simulink library "environmentLibrary"  (R2026a)
settings: Solver=ode45  EnableMultiTasking=on
undefined symbols (not defined in the file): decyear, initDate, leapyear
libraries: aerolibatmos2 x1, aerolibgravity2 x1
settings Model: Creator=The MathWorks, Inc.  LastModifiedBy=The MathWorks, Inc.
settings HardwareCC: ProdHWDeviceType=32-bit Generic

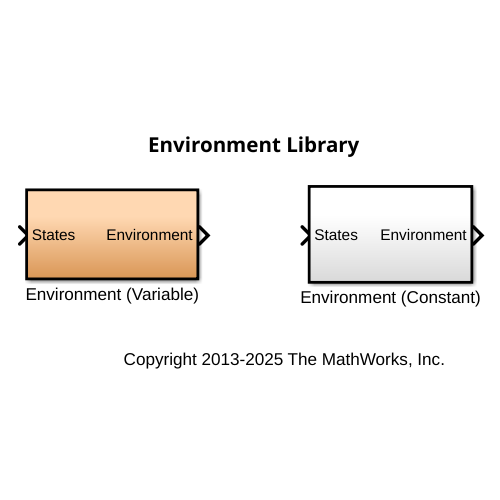
[thumbnail: Simulink's stored preview of the top-level diagram]
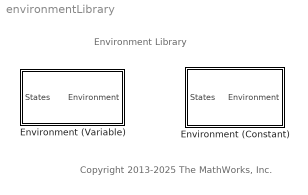
== system environmentLibrary ==
  note: Copyright 2013-2025 The MathWorks, Inc.
  note: Environment Library
  Environment (Constant) : Subsystem  TreatAsAtomicUnit=on
  Environment (Variable) : Subsystem  TreatAsAtomicUnit=on  VariantControl=Variants.Environment==1

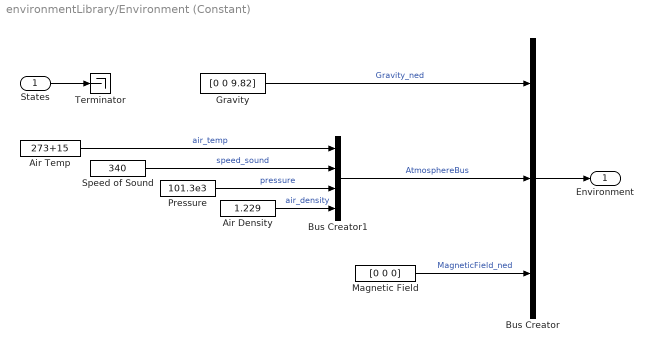
== system environmentLibrary/Environment (Constant) ==
  States : Inport  OutDataTypeStr=Bus: StatesBus
  Air Density : Constant  Value=1.229
  Air Temp : Constant  Value=273+15
  Bus Creator : BusCreator  Inputs=3  OutDataTypeStr=Bus: EnvironmentBus  NonVirtualBus=on
  Bus Creator1 : BusCreator  Inputs=4  OutDataTypeStr=Bus: AtmosphereBus  NonVirtualBus=on
  Gravity : Constant  Value=[0 0 9.82]
  Magnetic Field : Constant  Value=[0 0 0]
  Pressure : Constant  Value=101.3e3
  Speed of Sound : Constant  Value=340
  Terminator : Terminator
  Environment : Outport  VectorParamsAs1DForOutWhenUnconnected=off
  wires:
  Magnetic Field/1 -> Bus Creator/3  "MagneticField_ned"
  Bus Creator1/1 -> Bus Creator/2  "AtmosphereBus"
  Air Density/1 -> Bus Creator1/4  "air_density"
  Pressure/1 -> Bus Creator1/3  "pressure"
  Speed of Sound/1 -> Bus Creator1/2  "speed_sound"
  Air Temp/1 -> Bus Creator1/1  "air_temp"
  Bus Creator/1 -> Environment/1
  Gravity/1 -> Bus Creator/1  "Gravity_ned"
  States/1 -> Terminator/1

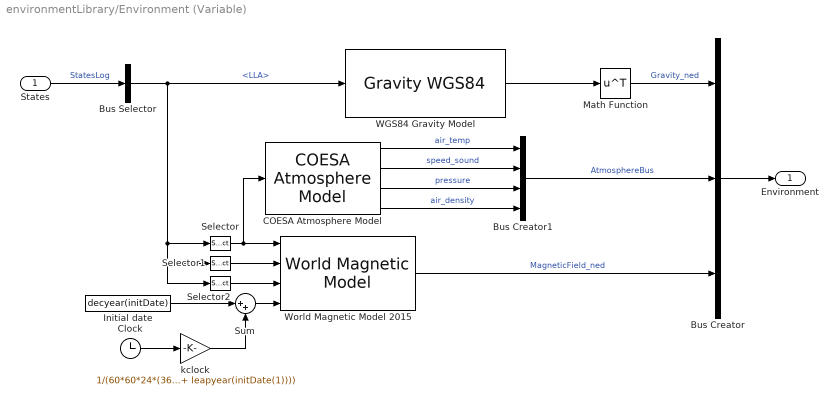
== system environmentLibrary/Environment (Variable) ==
  States : Inport  OutDataTypeStr=Bus: StatesBus
  Bus Creator : BusCreator  Inputs=3  OutDataTypeStr=Bus: EnvironmentBus  NonVirtualBus=on
  Bus Creator1 : BusCreator  Inputs=4  OutDataTypeStr=Bus: AtmosphereBus  NonVirtualBus=on
  Bus Selector : BusSelector  OutputSignals=LLA
  COESA Atmosphere Model : aerolibatmos2/COESA Atmosphere Model  units=Metric (MKS)  spec=1976 COESA-extended U.S. Standard Atmosphere  model=Profile  profile_var=High temperature  profile_percent=1%  profile_alt=5 km (16404 ft)  envelope_var=High temperature  envelope_percent=1%  action=Warning
  Clock : Clock
  Initial date : Constant  Value=decyear(initDate)
  Math Function : Math  Operator=transpose  SignedPower=on
  Selector : Selector  InputPortWidth=3  IndexOptions=Index vector (dialog)  Indices=[3]  OutputSizes=1
  Selector1 : Selector  InputPortWidth=3  IndexOptions=Index vector (dialog)  Indices=[1]  OutputSizes=1
  Selector2 : Selector  InputPortWidth=3  IndexOptions=Index vector (dialog)  Indices=[2]  OutputSizes=1
  Sum : Sum  Inputs=|++
  "WGS84 Gravity Model  " : GravityWGS84
  World Magnetic Model 2015 : aerolibgravity2/World Magnetic Model  model=WMM2015 V2 (2015-2020)  customFile='WMM2025.COF'  units=Metric (MKS)  time_in=on  month=January  day=1  year=2015  action=Error  h_out=off  dec_out=off  inc_out=off  ti_out=off
  kclock : Gain  Gain=1/(60*60*24*(365 + leapyear(initDate(1))))
  Environment : Outport  VectorParamsAs1DForOutWhenUnconnected=off
  wires:
  States/1 -> Bus Selector/1  "StatesLog"
  "WGS84 Gravity Model  "/1 -> Math Function/1
  Bus Creator/1 -> Environment/1
  COESA Atmosphere Model/1 -> Bus Creator1/1  "air_temp"
  COESA Atmosphere Model/2 -> Bus Creator1/2  "speed_sound"
  Bus Selector/1 -> "WGS84 Gravity Model  "/1, Selector2/1, Selector1/1, Selector/1  "<LLA>"
  COESA Atmosphere Model/3 -> Bus Creator1/3  "pressure"
  COESA Atmosphere Model/4 -> Bus Creator1/4  "air_density"
  Bus Creator1/1 -> Bus Creator/2  "AtmosphereBus"
  World Magnetic Model 2015/1 -> Bus Creator/3  "MagneticField_ned"
  Selector/1 -> World Magnetic Model 2015/1, COESA Atmosphere Model/1
  Selector1/1 -> World Magnetic Model 2015/2
  Selector2/1 -> World Magnetic Model 2015/3
  Math Function/1 -> Bus Creator/1  "Gravity_ned"
  Clock/1 -> kclock/1
  Initial date/1 -> Sum/1
  Sum/1 -> World Magnetic Model 2015/4
  kclock/1 -> Sum/2
